simulink model "dp7"  (R2026a)
settings: Solver=ode45  StopTime=120  RelTol=1e-6
InitFcn:
  | params7
values from neighbouring files (symbols this model uses):
  cpar = [kp kd ke dE tau_max Vin Vout]    [params.m]    (also in params7.m = [kE tau_sw tau_lqr Vin Vout kp_dn kd_dn])
  L1 = 0.5    [params.m]    (also in params7.m)
  L2 = 0.5    [params.m]    (also in params7.m = 0.4)
  p = [L1 W1 m1 L2 W2 m2 b1 b2 g]    [params.m]    (also in params7.m = [L1 lc1 m1 I1 L2 lc2 m2 I2 b1 b2 g])
  W1 = 0.05    [params.m]    (also in params7.m = 0.03)
  W2 = 0.04    [params.m]    (also in params7.m = 0.03)
  x0 = [0.01; 0; 0; 0]    [params.m]    (also in params7.m)
undefined symbols (not defined in the file or in its folder): K, P
settings Model: Creator=ern  LastModifiedBy=ern

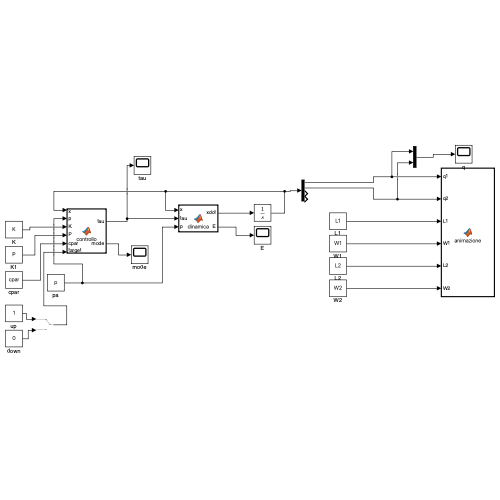
[thumbnail: Simulink's stored preview of the top-level diagram]
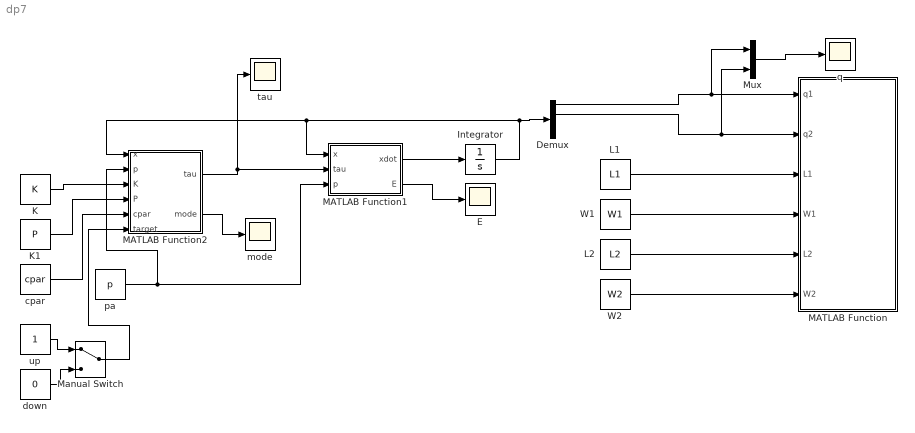
== system dp7 ==
  Demux : Demux
  E : Scope
      settings: ActiveDisplayYMinimum=-1  ActiveDisplayYMaximum=1
  Integrator : Integrator  InitialCondition=x0
  K : Constant  Value=K
  K1 : Constant  Value=P  VectorParams1D=off
  L1 : Constant  Value=L1
  L2 : Constant  Value=L2
  MATLAB Function : MATLAB Function  TreatAsAtomicUnit=on  SystemSampleTime=0.01
  MATLAB Function1 : MATLAB Function  TreatAsAtomicUnit=on
  MATLAB Function2 : MATLAB Function  TreatAsAtomicUnit=on  SystemSampleTime=0.001
  Manual Switch : ManualSwitch
  Mux : Mux  Inputs=2
  W1 : Constant  Value=W1
  W2 : Constant  Value=W2
  cpar : Constant  Value=cpar  VectorParams1D=off
  down : Constant  Value=0  VectorParams1D=off
  mode : Scope
      settings: ActiveDisplayYMinimum=-1  ActiveDisplayYMaximum=1  DataLoggingVariableName=ScopeData2
  pa : Constant  Value=p
  q : Scope
  tau : Scope
      settings: ActiveDisplayYMinimum=-1  ActiveDisplayYMaximum=1  DataLoggingVariableName=ScopeData3
  up : Constant  VectorParams1D=off
  wires:
  L1/1 -> MATLAB Function/3(L1)
  W1/1 -> MATLAB Function/4(W1)
  L2/1 -> MATLAB Function/5(L2)
  W2/1 -> MATLAB Function/6(W2)
  pa/1 -> MATLAB Function2/2(p), MATLAB Function1/3(p)
  MATLAB Function1/1(xdot) -> Integrator/1
  Integrator/1 -> MATLAB Function2/1(x), MATLAB Function1/1(x), Demux/1
  Demux/1 -> Mux/1, MATLAB Function/1(q1)
  Demux/2 -> Mux/2, MATLAB Function/2(q2)
  MATLAB Function1/2(E) -> E/1
  Mux/1 -> q/1
  MATLAB Function2/1(tau) -> tau/1, MATLAB Function1/2(tau)
  K/1 -> MATLAB Function2/3(K)
  K1/1 -> MATLAB Function2/4(P)
  cpar/1 -> MATLAB Function2/5(cpar)
  MATLAB Function2/2(mode) -> mode/1
  up/1 -> Manual Switch/1
  down/1 -> Manual Switch/2
  Manual Switch/1 -> MATLAB Function2/6(target)

== matlab function dp7/MATLAB Function1 ==
  data: x input; xdot output; tau input; p input; E output
function [xdot, E] = dinamica(x, tau, p)
L1 = p(1); lc1 = p(2); m1 = p(3); I1 = p(4);
L2 = p(5); lc2 = p(6); m2 = p(7); I2 = p(8);
b1 = p(9); b2  = p(10); g = p(11);

q1 = x(1); q2 = x(2); dq1 = x(3); dq2 = x(4);
c2 = cos(q2); s2 = sin(q2);

M11 = I1 + I2 + m1*lc1^2 + m2*(L1^2 + lc2^2 + 2*L1*lc2*c2);
M12 = I2 + m2*(lc2^2 + L1*lc2*c2);
M22 = I2 + m2*lc2^2;
M = [M11 M12; M12 M22];

h = m2*L1*lc2*s2;
C = [-h*(2*dq1*dq2 + dq2^2); h*dq1^2];
G = [(m1*lc1 + m2*L1)*g*sin(q1) + m2*lc2*g*sin(q1+q2);
      m2*lc2*g*sin(q1+q2)];
F = [b1*dq1; b2*dq2];

dq  = [dq1; dq2];
ddq = M \ ([tau; 0] - C - G - F);
xdot = [dq; ddq];

E = 0.5*dq.'*M*dq - m1*g*lc1*cos(q1) - m2*g*(L1*cos(q1) + lc2*cos(q1+q2));
end

== matlab function dp7/MATLAB Function ==
  data: q1 input; q2 input; L1 input; W1 input; L2 input; W2 input
function animazione(q1, q2, L1, W1, L2, W2)
coder.extrinsic('drawPendulum');
drawPendulum(q1, q2, L1, W1, L2, W2);
end

== matlab function dp7/MATLAB Function2 ==
  data: x input; tau output; p input; K input; P input; cpar input; mode output; target input
function [tau, mode] = controllo(x, p, K, P, cpar,target)
% Swing-up a pompaggio di energia puro + bilanciamento LQR
persistent m
if isempty(m), m = 0; end

L1 = p(1); lc1 = p(2); m1 = p(3); I1 = p(4);
L2 = p(5); lc2 = p(6); m2 = p(7); I2 = p(8); g = p(11);
kE = cpar(1); tau_sw = cpar(2); tau_lqr = cpar(3); Vin = cpar(4); Vout = cpar(5);
kp_dn = cpar(6); kd_dn = cpar(7);
q1 = x(1); q2 = x(2); dq1 = x(3); dq2 = x(4);

% Errore rispetto alla posizione invertita
e = [atan2(sin(q1-pi), cos(q1-pi)); atan2(sin(q2), cos(q2)); dq1; dq2];

% Commutazione con isteresi
V = e.'*P*e;
if target < 0.5
    m = 0;                          % target giù: niente LQR
elseif m == 0 && V < Vin
    m = 1;
elseif m == 1 && V > Vout
    m = 0;
end

if m == 1
    % --- Bilanciamento LQR ---
    tau = min(max(-K(:).'*e, -tau_lqr), tau_lqr);
else
    % --- Swing-up: pompaggio di energia ---
    c2 = cos(q2);
    M11 = I1 + I2 + m1*lc1^2 + m2*(L1^2 + lc2^2 + 2*L1*lc2*c2);
    M12 = I2 + m2*(lc2^2 + L1*lc2*c2);
    M22 = I2 + m2*lc2^2;
    dq = [dq1; dq2];
    E    = 0.5*dq.'*[M11 M12; M12 M22]*dq ...
           - m1*g*lc1*cos(q1) - m2*g*(L1*cos(q1) + lc2*cos(q1+q2));
    Etop = (m1*lc1 + m2*(L1 + lc2))*g;
    if target > 0.5
        tau = min(max(kE*(Etop - E)*dq1, -tau_sw), tau_sw);     % pompaggio verso l'alto
    else
        e1dn = atan2(sin(q1), cos(q1));                          % errore rispetto a q1 = 0
        tau  = min(max(-kp_dn*e1dn - kd_dn*dq1, -tau_sw), tau_sw); % discesa smorzata
    end
    %tau = min(max(kE*(Etop - E)*dq1, -tau_sw), tau_sw);
end
mode = m;
end
